simulink model "HarnessModel_BatteryHV"  (R2026a)
settings: Solver=daessc  StopTime=3600
PreLoadFcn:
  | setupHarness_BatteryHV
undefined symbols (not defined in the file or in its folder): Minus, Plus
libraries: nesl_utility x6, fl_lib x5
settings Model: Creator=isaacito  LastModifiedBy=isaacito
settings SimscapeCC: SimscapeNominalValues="[{\"value\":\"1\",\"unit\":\"A\"},{\"value\":\"1\",\"unit\":\"bar\"},{\"value\":\"1\",\"unit\":\"cm^2\"},{\"value\":\"1\",\"unit\":\"cm^3/s\"},{\"value\":\"1\",\"unit\":\"kJ/kg\"},{\"value\":\"1\",\"unit\":\"kW\"},{\"value\":\"1\",\"unit\":\"l\"},{\"value\":\"1\",\"unit\":\"N\"},{\"value\":\"1\",\"unit\":\"N*m\"},{\"value\":\"1\",\"unit\":\"V\"}]"  SimscapeLogSimulationStatistics=on  SimscapeLogLimitData=off  SimscapeLogDataHistory=5000.0

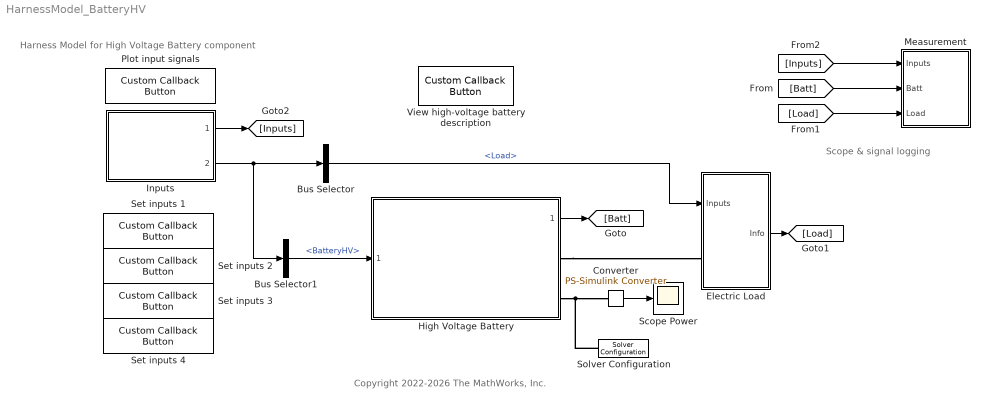
== system HarnessModel_BatteryHV ==
  note: Harness Model for High Voltage Battery component
  note: Copyright 2022-2026 The MathWorks, Inc.
  note: Scope & signal logging
  Bus Selector : BusSelector  OutputSignals=Load
  Bus Selector1 : BusSelector  OutputSignals=BatteryHV
  Converter : nesl_utility/PS-Simulink Converter  PhysicalDomain=network_engine_domain  SubClassName=ps_output  LeftPortType=input  RightPortType=output  PseudoPeriodic=off  Frequencies=[]  VectorFormat=inherit  Unit=kW  AffineConversion=off
  Electric Load : Subsystem
  High Voltage Battery : Subsystem  ReferencedSubsystem=BatteryHV_Basic_refsub
      settings: OpenFcn=|
      | % Look under mask:
      | open_system(gcb, "force")
  Inputs : Subsystem  ReferencedSubsystem=Inputs_BatteryHV_refsub
      settings: OpenFcn="open_system(gcb, \"force\")"
  Measurement : Subsystem
  Plot input signals : CustomCallbackButton  Configuration="{\"components\":[{\"name\":\"BackgroundImageComponent\",\"settings\":{\"image\":{\"size\":[0,0],\"src\":\"default\",\"srcOrientation\":\"Right\"},\"position\":[0,0,1,1]}},{\"name\":\"ButtonStateComponent\",\"settings\":{\"buttonType\":\"momentary\",\"clickFcn\":\"bevutil1.SignalUtil.plotLookupTable1DBlocks(bdroot+\\\"\\/Inputs\\\", Blocks=[\\\"\\/Load current\\\"; \\\"\\/Heat flow\\\"], DivisionType=\\\"InterpolationInterval\\\", InterpolationInterval=0.2)\",\"onValue\":1,\"position\":[0,0,1,1],\"pressDelay\":\"500\",\"pressFcn\":\"\",\"repeatInterval\":\"0\",\"states\":[{\"horizontalAlignment\":\"center\",\"image\":{\"position\":[0,0,1,1],\"size\":[1,1],\"src\":\"default\",\"srcOrientation\":\"Right\"},\"label\":{\"color\":[0.01176470588,0.01176470588,0.01176470588,1],\"icon\":{\"size\":[0,0],\"src\":\"default\",\"srcOrientation\":\"Right\"},\"iconOffset\":0,\"iconPlacement\":\"left\",\"opacity\":1,\"show\":true,\"text\":{\"content\":\"Plot inputs\",\"font\":\"Helvetica\"}},\"labelOffset\":[0,0],\"verticalAlignment\":\"middle\"},{\"horizontalAlignment\":\"center\",\"image\":{\"position\":[0,0,1,1],\"size\":[1,1],\"src\":\"default\",\"srcOrientation\":\"Right\"},\"label\":{\"color\":[0.01176470588,0.01176470588,0.01176470588,1],\"icon\":{\"size\":[0,0],\"src\":\"default\",\"srcOrientation\":\"Right\"},\"iconOffset\":0,\"iconPlacement\":\"left\",\"opacity\":1,\"show\":true,\"text\":{\"content\":\"Plot inputs\",\"font\":\"Helvetica\"}},\"labelOffset\":[0,0],\"verticalAlignment\":\"middle\"},{\"horizontalAlignment\":\"center\",\"image\":{\"position\":[0,0,1,1],\"size\":[1,1],\"src\":\"default\",\"srcOrientation\":\"Right\"},\"label\":{\"color\":[0.01176470588,0.01176470588,0.01176470588,1],\"icon\":{\"size\":[0,0],\"src\":\"default\",\"srcOrientation\":\"Right\"},\"iconOffset\":0,\"iconPlacement\":\"left\",\"opacity\":1,\"show\":true,\"text\":{\"content\":\"Plot inputs\",\"font\":\"Helvetica\"}},\"labelOffset\":[0,0],\"verticalAlignment\":\"middle\"},{\"horizontalAlignment\":\"center\",\"image\":{\"position\":[0,0,1,1],\"size\":[1,1],\"src\":\"default\",\"srcOrientation\":\"Right\"},\"label\":{\"color\":[0.01176470588,0.01176470588,0.01176470588,1],\"icon\":{\"size\":[0,0],\"src\":\"default\",\"srcOrientation\":\"Right\"},\"iconOffset\":0,\"iconPlacement\":\"left\",\"opacity\":1,\"show\":true,\"text\":{\"content\":\"Plot inputs\",\"font\":\"Helvetica\"}},\"labelOffset\":[0,0],\"verticalAlignment\":\"middle\"}]}},{\"name\":\"ForegroundImageComponent\",\"settings\":{\"image\":{\"size\":[0,0],\"src\":\"default\",\"srcOrientation\":\"Right\"},\"isForeground\":1,\"position\":[0,0,1,1]}}],\"derived\":{\"blockParameters\":{\"AutoActivate\":true,\"ButtonText\":\"Plot inputs\",\"ButtonType\":\"Momentary\",\"ClickFcn\":\"bevutil1.SignalUtil.plotLookupTable1DBlocks(bdroot+\\\"\\/Inputs\\\", Blocks=[\\\"\\/Load current\\\"; \\\"\\/Heat flow\\\"], DivisionType=\\\"InterpolationInterval\\\", InterpolationInterval=0.2)\",\"OnValue\":1,\"PressDelay\":\"500\",\"PressFcn\":\"\",\"RepeatInterval\":\"0\",\"fixedAspectRatio\":\"off\"}},\"settings\":{\"BindingType\":\"standalone\",\"autoActivate\":true,\"backgroundColor\":[244,244,244,1],\"backgroundOffset\":0.2,\"backgroundOpacity\":1,\"fixedAspectRatio\":\"off\",\"foregroundColor\":[0.01176470588,0.01176470588,0.01176470588,1],\"migratedFromLegacy\":true,\"useBackgroundColor\":true,\"variant\":\"callback\",\"version\":\"R2025a\"},\"type\":\"Button\"}"  CustomBackgroundColor="{\"color\":[0.9568627451,0.9568627451,0.9568627451],\"show\":true}"
  Scope Power : Scope
      settings: ActiveDisplayYMinimum=-3.3202715007040107  ActiveDisplayYMaximum=7.2203137029230895
  Set inputs 1 : CustomCallbackButton  Configuration="{\"components\":[{\"name\":\"BackgroundImageComponent\",\"settings\":{\"image\":{\"size\":[0,0],\"src\":\"default\",\"srcOrientation\":\"Right\"},\"position\":[0,0,1,1]}},{\"name\":\"ButtonStateComponent\",\"settings\":{\"buttonType\":\"momentary\",\"clickFcn\":\"BatteryHV_Basic_params\\nset_param(gcs, StopTime=\\\"3600\\\")\\n\\ndisp(\\\"Loading inputs: <a href=\\\"\\\"matlab:edit('LoadInputs_BatteryHV_Constant')\\\"\\\">Constant<\\/a>\\\")\\nLoadInputs_BatteryHV_Constant\\n\",\"onValue\":1,\"position\":[0,0,1,1],\"pressDelay\":\"500\",\"pressFcn\":\"\",\"repeatInterval\":\"0\",\"states\":[{\"horizontalAlignment\":\"center\",\"image\":{\"position\":[0,0,1,1],\"size\":[1,1],\"src\":\"default\",\"srcOrientation\":\"Right\"},\"label\":{\"color\":[0.01176470588,0.01176470588,0.01176470588,1],\"icon\":{\"size\":[0,0],\"src\":\"default\",\"srcOrientation\":\"Right\"},\"iconOffset\":0,\"iconPlacement\":\"left\",\"opacity\":1,\"show\":true,\"text\":{\"content\":\"Constant\",\"font\":\"Helvetica\"}},\"labelOffset\":[0,0],\"verticalAlignment\":\"middle\"},{\"horizontalAlignment\":\"center\",\"image\":{\"position\":[0,0,1,1],\"size\":[1,1],\"src\":\"default\",\"srcOrientation\":\"Right\"},\"label\":{\"color\":[0.01176470588,0.01176470588,0.01176470588,1],\"icon\":{\"size\":[0,0],\"src\":\"default\",\"srcOrientation\":\"Right\"},\"iconOffset\":0,\"iconPlacement\":\"left\",\"opacity\":1,\"show\":true,\"text\":{\"content\":\"Constant\",\"font\":\"Helvetica\"}},\"labelOffset\":[0,0],\"verticalAlignment\":\"middle\"},{\"horizontalAlignment\":\"center\",\"image\":{\"position\":[0,0,1,1],\"size\":[1,1],\"src\":\"default\",\"srcOrientation\":\"Right\"},\"label\":{\"color\":[0.01176470588,0.01176470588,0.01176470588,1],\"icon\":{\"size\":[0,0],\"src\":\"default\",\"srcOrientation\":\"Right\"},\"iconOffset\":0,\"iconPlacement\":\"left\",\"opacity\":1,\"show\":true,\"text\":{\"content\":\"Constant\",\"font\":\"Helvetica\"}},\"labelOffset\":[0,0],\"verticalAlignment\":\"middle\"},{\"horizontalAlignment\":\"center\",\"image\":{\"position\":[0,0,1,1],\"size\":[1,1],\"src\":\"default\",\"srcOrientation\":\"Right\"},\"label\":{\"color\":[0.01176470588,0.01176470588,0.01176470588,1],\"icon\":{\"size\":[0,0],\"src\":\"default\",\"srcOrientation\":\"Right\"},\"iconOffset\":0,\"iconPlacement\":\"left\",\"opacity\":1,\"show\":true,\"text\":{\"content\":\"Constant\",\"font\":\"Helvetica\"}},\"labelOffset\":[0,0],\"verticalAlignment\":\"middle\"}]}},{\"name\":\"ForegroundImageComponent\",\"settings\":{\"image\":{\"size\":[0,0],\"src\":\"default\",\"srcOrientation\":\"Right\"},\"isForeground\":1,\"position\":[0,0,1,1]}}],\"derived\":{\"blockParameters\":{\"AutoActivate\":true,\"ButtonText\":\"Constant\",\"ButtonType\":\"Momentary\",\"ClickFcn\":\"BatteryHV_Basic_params\\nset_param(gcs, StopTime=\\\"3600\\\")\\n\\ndisp(\\\"Loading inputs: <a href=\\\"\\\"matlab:edit('LoadInputs_BatteryHV_Constant')\\\"\\\">Constant<\\/a>\\\")\\nLoadInputs_BatteryHV_Constant\\n\",\"OnValue\":1,\"PressDelay\":\"500\",\"PressFcn\":\"\",\"RepeatInterval\":\"0\",\"fixedAspectRatio\":\"off\"}},\"settings\":{\"BindingType\":\"standalone\",\"autoActivate\":true,\"backgroundColor\":[244,244,244,1],\"backgroundOffset\":0.2,\"backgroundOpacity\":1,\"fixedAspectRatio\":\"off\",\"foregroundColor\":[0.01176470588,0.01176470588,0.01176470588,1],\"migratedFromLegacy\":true,\"useBackgroundColor\":true,\"variant\":\"callback\",\"version\":\"R2025a\"},\"type\":\"Button\"}"  CustomBackgroundColor="{\"color\":[0.9568627451,0.9568627451,0.9568627451],\"show\":true}"
  Set inputs 2 : CustomCallbackButton  Configuration="{\"components\":[{\"name\":\"BackgroundImageComponent\",\"settings\":{\"image\":{\"size\":[0,0],\"src\":\"default\",\"srcOrientation\":\"Right\"},\"position\":[0,0,1,1]}},{\"name\":\"ButtonStateComponent\",\"settings\":{\"buttonType\":\"momentary\",\"clickFcn\":\"BatteryHV_Basic_params\\nset_param(gcs, StopTime=\\\"3600\\\")\\n\\ndisp(\\\"Loading inputs: <a href=\\\"\\\"matlab:edit('LoadInputs_BatteryHV_Charge')\\\"\\\">Charge<\\/a>\\\")\\nLoadInputs_BatteryHV_Charge\\n\",\"onValue\":1,\"position\":[0,0,1,1],\"pressDelay\":\"500\",\"pressFcn\":\"\",\"repeatInterval\":\"0\",\"states\":[{\"horizontalAlignment\":\"center\",\"image\":{\"position\":[0,0,1,1],\"size\":[1,1],\"src\":\"default\",\"srcOrientation\":\"Right\"},\"label\":{\"color\":[0.01176470588,0.01176470588,0.01176470588,1],\"icon\":{\"size\":[0,0],\"src\":\"default\",\"srcOrientation\":\"Right\"},\"iconOffset\":0,\"iconPlacement\":\"left\",\"opacity\":1,\"show\":true,\"text\":{\"content\":\"Charge\",\"font\":\"Helvetica\"}},\"labelOffset\":[0,0],\"verticalAlignment\":\"middle\"},{\"horizontalAlignment\":\"center\",\"image\":{\"position\":[0,0,1,1],\"size\":[1,1],\"src\":\"default\",\"srcOrientation\":\"Right\"},\"label\":{\"color\":[0.01176470588,0.01176470588,0.01176470588,1],\"icon\":{\"size\":[0,0],\"src\":\"default\",\"srcOrientation\":\"Right\"},\"iconOffset\":0,\"iconPlacement\":\"left\",\"opacity\":1,\"show\":true,\"text\":{\"content\":\"Charge\",\"font\":\"Helvetica\"}},\"labelOffset\":[0,0],\"verticalAlignment\":\"middle\"},{\"horizontalAlignment\":\"center\",\"image\":{\"position\":[0,0,1,1],\"size\":[1,1],\"src\":\"default\",\"srcOrientation\":\"Right\"},\"label\":{\"color\":[0.01176470588,0.01176470588,0.01176470588,1],\"icon\":{\"size\":[0,0],\"src\":\"default\",\"srcOrientation\":\"Right\"},\"iconOffset\":0,\"iconPlacement\":\"left\",\"opacity\":1,\"show\":true,\"text\":{\"content\":\"Charge\",\"font\":\"Helvetica\"}},\"labelOffset\":[0,0],\"verticalAlignment\":\"middle\"},{\"horizontalAlignment\":\"center\",\"image\":{\"position\":[0,0,1,1],\"size\":[1,1],\"src\":\"default\",\"srcOrientation\":\"Right\"},\"label\":{\"color\":[0.01176470588,0.01176470588,0.01176470588,1],\"icon\":{\"size\":[0,0],\"src\":\"default\",\"srcOrientation\":\"Right\"},\"iconOffset\":0,\"iconPlacement\":\"left\",\"opacity\":1,\"show\":true,\"text\":{\"content\":\"Charge\",\"font\":\"Helvetica\"}},\"labelOffset\":[0,0],\"verticalAlignment\":\"middle\"}]}},{\"name\":\"ForegroundImageComponent\",\"settings\":{\"image\":{\"size\":[0,0],\"src\":\"default\",\"srcOrientation\":\"Right\"},\"isForeground\":1,\"position\":[0,0,1,1]}}],\"derived\":{\"blockParameters\":{\"AutoActivate\":true,\"ButtonText\":\"Charge\",\"ButtonType\":\"Momentary\",\"ClickFcn\":\"BatteryHV_Basic_params\\nset_param(gcs, StopTime=\\\"3600\\\")\\n\\ndisp(\\\"Loading inputs: <a href=\\\"\\\"matlab:edit('LoadInputs_BatteryHV_Charge')\\\"\\\">Charge<\\/a>\\\")\\nLoadInputs_BatteryHV_Charge\\n\",\"OnValue\":1,\"PressDelay\":\"500\",\"PressFcn\":\"\",\"RepeatInterval\":\"0\",\"fixedAspectRatio\":\"off\"}},\"settings\":{\"BindingType\":\"standalone\",\"autoActivate\":true,\"backgroundColor\":[244,244,244,1],\"backgroundOffset\":0.2,\"backgroundOpacity\":1,\"fixedAspectRatio\":\"off\",\"foregroundColor\":[0.01176470588,0.01176470588,0.01176470588,1],\"migratedFromLegacy\":true,\"useBackgroundColor\":true,\"variant\":\"callback\",\"version\":\"R2025a\"},\"type\":\"Button\"}"  CustomBackgroundColor="{\"color\":[0.9568627451,0.9568627451,0.9568627451],\"show\":true}"
  Set inputs 3 : CustomCallbackButton  Configuration="{\"components\":[{\"name\":\"BackgroundImageComponent\",\"settings\":{\"image\":{\"size\":[0,0],\"src\":\"default\",\"srcOrientation\":\"Right\"},\"position\":[0,0,1,1]}},{\"name\":\"ButtonStateComponent\",\"settings\":{\"buttonType\":\"momentary\",\"clickFcn\":\"BatteryHV_Basic_params\\nset_param(gcs, StopTime=\\\"3600\\\")\\n\\ndisp(\\\"Loading inputs: <a href=\\\"\\\"matlab:edit('LoadInputs_BatteryHV_Discharge')\\\"\\\">Discharge<\\/a>\\\")\\nLoadInputs_BatteryHV_Discharge\\n\",\"onValue\":1,\"position\":[0,0,1,1],\"pressDelay\":\"500\",\"pressFcn\":\"\",\"repeatInterval\":\"0\",\"states\":[{\"horizontalAlignment\":\"center\",\"image\":{\"position\":[0,0,1,1],\"size\":[1,1],\"src\":\"default\",\"srcOrientation\":\"Right\"},\"label\":{\"color\":[0.01176470588,0.01176470588,0.01176470588,1],\"icon\":{\"size\":[0,0],\"src\":\"default\",\"srcOrientation\":\"Right\"},\"iconOffset\":0,\"iconPlacement\":\"left\",\"opacity\":1,\"show\":true,\"text\":{\"content\":\"Discharge\",\"font\":\"Helvetica\"}},\"labelOffset\":[0,0],\"verticalAlignment\":\"middle\"},{\"horizontalAlignment\":\"center\",\"image\":{\"position\":[0,0,1,1],\"size\":[1,1],\"src\":\"default\",\"srcOrientation\":\"Right\"},\"label\":{\"color\":[0.01176470588,0.01176470588,0.01176470588,1],\"icon\":{\"size\":[0,0],\"src\":\"default\",\"srcOrientation\":\"Right\"},\"iconOffset\":0,\"iconPlacement\":\"left\",\"opacity\":1,\"show\":true,\"text\":{\"content\":\"Discharge\",\"font\":\"Helvetica\"}},\"labelOffset\":[0,0],\"verticalAlignment\":\"middle\"},{\"horizontalAlignment\":\"center\",\"image\":{\"position\":[0,0,1,1],\"size\":[1,1],\"src\":\"default\",\"srcOrientation\":\"Right\"},\"label\":{\"color\":[0.01176470588,0.01176470588,0.01176470588,1],\"icon\":{\"size\":[0,0],\"src\":\"default\",\"srcOrientation\":\"Right\"},\"iconOffset\":0,\"iconPlacement\":\"left\",\"opacity\":1,\"show\":true,\"text\":{\"content\":\"Discharge\",\"font\":\"Helvetica\"}},\"labelOffset\":[0,0],\"verticalAlignment\":\"middle\"},{\"horizontalAlignment\":\"center\",\"image\":{\"position\":[0,0,1,1],\"size\":[1,1],\"src\":\"default\",\"srcOrientation\":\"Right\"},\"label\":{\"color\":[0.01176470588,0.01176470588,0.01176470588,1],\"icon\":{\"size\":[0,0],\"src\":\"default\",\"srcOrientation\":\"Right\"},\"iconOffset\":0,\"iconPlacement\":\"left\",\"opacity\":1,\"show\":true,\"text\":{\"content\":\"Discharge\",\"font\":\"Helvetica\"}},\"labelOffset\":[0,0],\"verticalAlignment\":\"middle\"}]}},{\"name\":\"ForegroundImageComponent\",\"settings\":{\"image\":{\"size\":[0,0],\"src\":\"default\",\"srcOrientation\":\"Right\"},\"isForeground\":1,\"position\":[0,0,1,1]}}],\"derived\":{\"blockParameters\":{\"AutoActivate\":true,\"ButtonText\":\"Discharge\",\"ButtonType\":\"Momentary\",\"ClickFcn\":\"BatteryHV_Basic_params\\nset_param(gcs, StopTime=\\\"3600\\\")\\n\\ndisp(\\\"Loading inputs: <a href=\\\"\\\"matlab:edit('LoadInputs_BatteryHV_Discharge')\\\"\\\">Discharge<\\/a>\\\")\\nLoadInputs_BatteryHV_Discharge\\n\",\"OnValue\":1,\"PressDelay\":\"500\",\"PressFcn\":\"\",\"RepeatInterval\":\"0\",\"fixedAspectRatio\":\"off\"}},\"settings\":{\"BindingType\":\"standalone\",\"autoActivate\":true,\"backgroundColor\":[244,244,244,1],\"backgroundOffset\":0.2,\"backgroundOpacity\":1,\"fixedAspectRatio\":\"off\",\"foregroundColor\":[0.01176470588,0.01176470588,0.01176470588,1],\"migratedFromLegacy\":true,\"useBackgroundColor\":true,\"variant\":\"callback\",\"version\":\"R2025a\"},\"type\":\"Button\"}"  CustomBackgroundColor="{\"color\":[0.9568627451,0.9568627451,0.9568627451],\"show\":true}"
  Set inputs 4 : CustomCallbackButton  Configuration="{\"components\":[{\"name\":\"BackgroundImageComponent\",\"settings\":{\"image\":{\"size\":[0,0],\"src\":\"default\",\"srcOrientation\":\"Right\"},\"position\":[0,0,1,1]}},{\"name\":\"ButtonStateComponent\",\"settings\":{\"buttonType\":\"momentary\",\"clickFcn\":\"BatteryHV_Basic_params\\n\\ndisp(\\\"Loading inputs: <a href=\\\"\\\"matlab:edit('LoadInputs_BatteryHV_Random')\\\"\\\">Random<\\/a>\\\")\\nLoadInputs_BatteryHV_Random\\n\\ntmp_stop_time = get_param(bdroot+\\\"\\/Inputs\\/Load current\\\", \\\"value@BreakpointsForDimension1\\\");\\nset_param(bdroot, StopTime=num2str(tmp_stop_time(end)) )\\ndisp(\\\"Stop time: \\\" + tmp_stop_time(end))\\nclear tmp_stop_time\\n\",\"onValue\":1,\"position\":[0,0,1,1],\"pressDelay\":\"500\",\"pressFcn\":\"\",\"repeatInterval\":\"0\",\"states\":[{\"horizontalAlignment\":\"center\",\"image\":{\"position\":[0,0,1,1],\"size\":[1,1],\"src\":\"default\",\"srcOrientation\":\"Right\"},\"label\":{\"color\":[0.01176470588,0.01176470588,0.01176470588,1],\"icon\":{\"size\":[0,0],\"src\":\"default\",\"srcOrientation\":\"Right\"},\"iconOffset\":0,\"iconPlacement\":\"left\",\"opacity\":1,\"show\":true,\"text\":{\"content\":\"Random\",\"font\":\"Helvetica\"}},\"labelOffset\":[0,0],\"verticalAlignment\":\"middle\"},{\"horizontalAlignment\":\"center\",\"image\":{\"position\":[0,0,1,1],\"size\":[1,1],\"src\":\"default\",\"srcOrientation\":\"Right\"},\"label\":{\"color\":[0.01176470588,0.01176470588,0.01176470588,1],\"icon\":{\"size\":[0,0],\"src\":\"default\",\"srcOrientation\":\"Right\"},\"iconOffset\":0,\"iconPlacement\":\"left\",\"opacity\":1,\"show\":true,\"text\":{\"content\":\"Random\",\"font\":\"Helvetica\"}},\"labelOffset\":[0,0],\"verticalAlignment\":\"middle\"},{\"horizontalAlignment\":\"center\",\"image\":{\"position\":[0,0,1,1],\"size\":[1,1],\"src\":\"default\",\"srcOrientation\":\"Right\"},\"label\":{\"color\":[0.01176470588,0.01176470588,0.01176470588,1],\"icon\":{\"size\":[0,0],\"src\":\"default\",\"srcOrientation\":\"Right\"},\"iconOffset\":0,\"iconPlacement\":\"left\",\"opacity\":1,\"show\":true,\"text\":{\"content\":\"Random\",\"font\":\"Helvetica\"}},\"labelOffset\":[0,0],\"verticalAlignment\":\"middle\"},{\"horizontalAlignment\":\"center\",\"image\":{\"position\":[0,0,1,1],\"size\":[1,1],\"src\":\"default\",\"srcOrientation\":\"Right\"},\"label\":{\"color\":[0.01176470588,0.01176470588,0.01176470588,1],\"icon\":{\"size\":[0,0],\"src\":\"default\",\"srcOrientation\":\"Right\"},\"iconOffset\":0,\"iconPlacement\":\"left\",\"opacity\":1,\"show\":true,\"text\":{\"content\":\"Random\",\"font\":\"Helvetica\"}},\"labelOffset\":[0,0],\"verticalAlignment\":\"middle\"}]}},{\"name\":\"ForegroundImageComponent\",\"settings\":{\"image\":{\"size\":[0,0],\"src\":\"default\",\"srcOrientation\":\"Right\"},\"isForeground\":1,\"position\":[0,0,1,1]}}],\"derived\":{\"blockParameters\":{\"AutoActivate\":true,\"ButtonText\":\"Random\",\"ButtonType\":\"Momentary\",\"ClickFcn\":\"BatteryHV_Basic_params\\n\\ndisp(\\\"Loading inputs: <a href=\\\"\\\"matlab:edit('LoadInputs_BatteryHV_Random')\\\"\\\">Random<\\/a>\\\")\\nLoadInputs_BatteryHV_Random\\n\\ntmp_stop_time = get_param(bdroot+\\\"\\/Inputs\\/Load current\\\", \\\"value@BreakpointsForDimension1\\\");\\nset_param(bdroot, StopTime=num2str(tmp_stop_time(end)) )\\ndisp(\\\"Stop time: \\\" + tmp_stop_time(end))\\nclear tmp_stop_time\\n\",\"OnValue\":1,\"PressDelay\":\"500\",\"PressFcn\":\"\",\"RepeatInterval\":\"0\",\"fixedAspectRatio\":\"off\"}},\"settings\":{\"BindingType\":\"standalone\",\"autoActivate\":true,\"backgroundColor\":[244,244,244,1],\"backgroundOffset\":0.2,\"backgroundOpacity\":1,\"fixedAspectRatio\":\"off\",\"foregroundColor\":[0.01176470588,0.01176470588,0.01176470588,1],\"migratedFromLegacy\":true,\"useBackgroundColor\":true,\"variant\":\"callback\",\"version\":\"R2025a\"},\"type\":\"Button\"}"  CustomBackgroundColor="{\"color\":[0.9568627451,0.9568627451,0.9568627451],\"show\":true}"
  Solver Configuration : nesl_utility/Solver Configuration  PhysicalDomain=network_engine_domain  SubClassName=solver  LeftPortType=input  RightPortType=generic  Tones=[]  Harmonics=[]  SimulateNoise=off  Profile=off  UseLocalSampling=off  EnableSwitchedLinearOptims=on  FrequencyDomain=off  UseCCode=off  RelTol=0.001  AbsTol=0.001  MinStep=1e-09  ToWorkspace=off  RevertToSquareIcSolve=off  NumHomotopyIterations=100  PhasorMode=off  PhasorModeNumHarmonics=1  ConsistencySolver=NEWTON_FTOL  CanonicalOrdering=UNORDERED  OptimizeIntermediates=UNOPTIMIZED  IndexReductionMethod=DerivativeReplacement  DoDC=off  ResidualTolerance=1e-09  ConsistencyTolSource=GLOBAL  ConsistencyAbsTol=0.001  ConsistencyRelTol=0.001  ConsistencyTolFactor=0.001  UseLocalSolver=off  LocalSolverChoice=NE_BACKWARD_EULER_ADVANCER  ResolveIndetEquations=on  FunctionEvalNumThread=1  LocalSolverSampleTime=0.001  DoFixedCost=off  MaxNonlinIter=3  MaxModeIter=2  ComputeImpulses=off  ImpulseIterations=2  LinearAlgebra=auto  LinearAlgebraNumThread=0  EquationFormulation=NE_TIME_EF  DelaysMemoryBudget=1024  AutomaticFiltering=on  FilteringTimeConstant=0.001  PartitionStorageMethod=AS_NEEDED  PartitionMemoryBudget=1024  PartitionMethod=ROBUST  MultibodyUseLocalSolver=off  MultibodyLocalSolverChoice=ODE1  MultibodyLocalSolverSampleTime=0.001
      settings: AttributesFormatString=Local solver: %<UseLocalSolver>
  View high-voltage battery description : CustomCallbackButton  Configuration="{\"components\":[{\"name\":\"BackgroundImageComponent\",\"settings\":{\"image\":{\"size\":[0,0],\"src\":\"default\",\"srcOrientation\":\"Right\"},\"position\":[0,0,1,1]}},{\"name\":\"ButtonStateComponent\",\"settings\":{\"buttonType\":\"momentary\",\"clickFcn\":\"web(\\\"BatteryHV_Description.html\\\")\",\"onValue\":1,\"position\":[0,0,1,1],\"pressDelay\":\"500\",\"pressFcn\":\"\",\"repeatInterval\":\"0\",\"states\":[{\"horizontalAlignment\":\"center\",\"image\":{\"position\":[0,0,1,1],\"size\":[1,1],\"src\":\"default\",\"srcOrientation\":\"Right\"},\"label\":{\"color\":[0.01176470588,0.01176470588,0.01176470588,1],\"icon\":{\"size\":[0,0],\"src\":\"default\",\"srcOrientation\":\"Right\"},\"iconOffset\":0,\"iconPlacement\":\"left\",\"opacity\":1,\"show\":true,\"text\":{\"content\":\"Open page\",\"font\":\"Helvetica\"}},\"labelOffset\":[0,0],\"verticalAlignment\":\"middle\"},{\"horizontalAlignment\":\"center\",\"image\":{\"position\":[0,0,1,1],\"size\":[1,1],\"src\":\"default\",\"srcOrientation\":\"Right\"},\"label\":{\"color\":[0.01176470588,0.01176470588,0.01176470588,1],\"icon\":{\"size\":[0,0],\"src\":\"default\",\"srcOrientation\":\"Right\"},\"iconOffset\":0,\"iconPlacement\":\"left\",\"opacity\":1,\"show\":true,\"text\":{\"content\":\"Open page\",\"font\":\"Helvetica\"}},\"labelOffset\":[0,0],\"verticalAlignment\":\"middle\"},{\"horizontalAlignment\":\"center\",\"image\":{\"position\":[0,0,1,1],\"size\":[1,1],\"src\":\"default\",\"srcOrientation\":\"Right\"},\"label\":{\"color\":[0.01176470588,0.01176470588,0.01176470588,1],\"icon\":{\"size\":[0,0],\"src\":\"default\",\"srcOrientation\":\"Right\"},\"iconOffset\":0,\"iconPlacement\":\"left\",\"opacity\":1,\"show\":true,\"text\":{\"content\":\"Open page\",\"font\":\"Helvetica\"}},\"labelOffset\":[0,0],\"verticalAlignment\":\"middle\"},{\"horizontalAlignment\":\"center\",\"image\":{\"position\":[0,0,1,1],\"size\":[1,1],\"src\":\"default\",\"srcOrientation\":\"Right\"},\"label\":{\"color\":[0.01176470588,0.01176470588,0.01176470588,1],\"icon\":{\"size\":[0,0],\"src\":\"default\",\"srcOrientation\":\"Right\"},\"iconOffset\":0,\"iconPlacement\":\"left\",\"opacity\":1,\"show\":true,\"text\":{\"content\":\"Open page\",\"font\":\"Helvetica\"}},\"labelOffset\":[0,0],\"verticalAlignment\":\"middle\"}]}},{\"name\":\"ForegroundImageComponent\",\"settings\":{\"image\":{\"size\":[0,0],\"src\":\"default\",\"srcOrientation\":\"Right\"},\"isForeground\":1,\"position\":[0,0,1,1]}}],\"derived\":{\"blockParameters\":{\"AutoActivate\":true,\"ButtonText\":\"Open page\",\"ButtonType\":\"Momentary\",\"ClickFcn\":\"web(\\\"BatteryHV_Description.html\\\")\",\"OnValue\":1,\"PressDelay\":\"500\",\"PressFcn\":\"\",\"RepeatInterval\":\"0\",\"fixedAspectRatio\":\"off\"}},\"settings\":{\"BindingType\":\"standalone\",\"autoActivate\":true,\"backgroundColor\":[244,244,244,1],\"backgroundOffset\":0.2,\"backgroundOpacity\":1,\"fixedAspectRatio\":\"off\",\"foregroundColor\":[0.01176470588,0.01176470588,0.01176470588,1],\"migratedFromLegacy\":true,\"useBackgroundColor\":true,\"variant\":\"callback\",\"version\":\"R2025a\"},\"type\":\"Button\"}"  CustomBackgroundColor="{\"color\":[0.9568627450980393,0.9568627450980393,0.9568627450980393],\"show\":true}"
  wires:
  High Voltage Battery/1 -> [Batt]
  [Batt] -> Measurement/2(Batt)
  Electric Load/1(Info) -> [Load]
  [Load] -> Measurement/3(Load)
  [Inputs] -> Measurement/1(Inputs)
  Inputs/1 -> [Inputs]
  Inputs/2 -> Bus Selector/1, Bus Selector1/1
  Bus Selector/1 -> Electric Load/1(Inputs)  "<Load>"
  Bus Selector1/1 -> High Voltage Battery/1  "<BatteryHV>"
  Converter/1 -> Scope Power/1
  connections:
  High Voltage Battery/RConn1 -- Electric Load/LConn1
  High Voltage Battery/RConn2 -- Solver Configuration/RConn1 -- Converter/LConn1

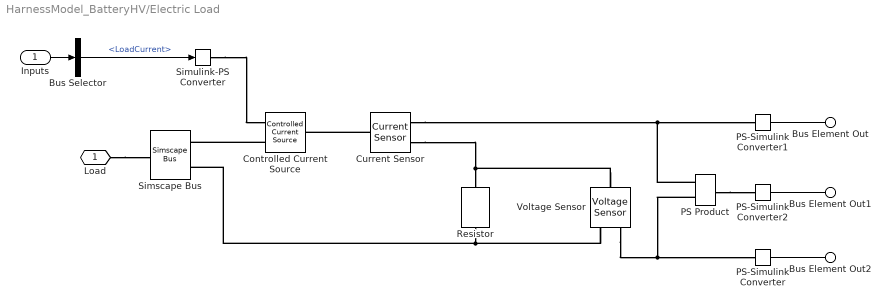
== system HarnessModel_BatteryHV/Electric Load ==
  Inputs : Inport
  Bus Selector : BusSelector  OutputSignals=LoadCurrent
  Controlled Current Source : fl_lib/Electrical/Electrical Sources/Controlled Current Source
  Current Sensor : fl_lib/Electrical/Electrical Sensors/Current Sensor
  PS Product : fl_lib/Physical Signals/Functions/PS Product
  PS-Simulink Converter : nesl_utility/PS-Simulink Converter  PhysicalDomain=network_engine_domain  SubClassName=ps_output  LeftPortType=input  RightPortType=output  PseudoPeriodic=off  Frequencies=[]  VectorFormat=inherit  Unit=V  AffineConversion=off
  PS-Simulink Converter1 : nesl_utility/PS-Simulink Converter  PhysicalDomain=network_engine_domain  SubClassName=ps_output  LeftPortType=input  RightPortType=output  PseudoPeriodic=off  Frequencies=[]  VectorFormat=inherit  Unit=A  AffineConversion=off
  PS-Simulink Converter2 : nesl_utility/PS-Simulink Converter  PhysicalDomain=network_engine_domain  SubClassName=ps_output  LeftPortType=input  RightPortType=output  PseudoPeriodic=off  Frequencies=[]  VectorFormat=inherit  Unit=kW  AffineConversion=off
  Resistor : fl_lib/Electrical/Electrical Elements/Resistor  R=1 Ohm  i_specify=off  i_priority=None  i=0 A  i_nominal_specify=off  i_nominal_value=1  i_nominal_unit=A  v_specify=off  v_priority=None  v=0 V  v_nominal_specify=off  v_nominal_value=1  v_nominal_unit=V
  Simscape Bus : SimscapeBus  HierarchyStrings=Plus;Minus  ConnectionType=Bus: Bus_HighVoltage
  Simulink-PS Converter : nesl_utility/Simulink-PS Converter  PhysicalDomain=network_engine_domain  SubClassName=ps_input  LeftPortType=input  RightPortType=output  PseudoPeriodic=off  Frequencies=[]  NoiseDistribution=none  NoiseParameters=[]  Unit=A  AffineConversion=off  FilteringAndDerivatives=provide  SimscapeFilterOrder=1  InputFilterTimeConstant=0.001  UdotUserProvided=0
  Voltage Sensor : fl_lib/Electrical/Electrical Sensors/Voltage Sensor
  Load : PMIOPort  Side=Left
  Bus Element Out : Outport  PortName=Info  Element=Curr
  Bus Element Out1 : Outport  PortName=Info  Element=Pwr
  Bus Element Out2 : Outport  PortName=Info  Element=V
  wires:
  PS-Simulink Converter1/1 -> Bus Element Out/1
  PS-Simulink Converter2/1 -> Bus Element Out1/1
  PS-Simulink Converter/1 -> Bus Element Out2/1
  Inputs/1 -> Bus Selector/1
  Bus Selector/1 -> Simulink-PS Converter/1  "<LoadCurrent>"
  connections:
  Load/RConn1 -- Simscape Bus/RConn1
  Controlled Current Source/RConn2 -- Simscape Bus/LConn1
  Resistor/RConn1 -- Voltage Sensor/RConn2 -- Simscape Bus/LConn2
  Simulink-PS Converter/RConn1 -- Controlled Current Source/RConn1
  Current Sensor/LConn1 -- Controlled Current Source/LConn1
  Current Sensor/RConn2 -- Voltage Sensor/LConn1 -- Resistor/LConn1
  Voltage Sensor/RConn1 -- PS Product/LConn2 -- PS-Simulink Converter/LConn1
  Current Sensor/RConn1 -- PS Product/LConn1 -- PS-Simulink Converter1/LConn1
  PS Product/RConn1 -- PS-Simulink Converter2/LConn1

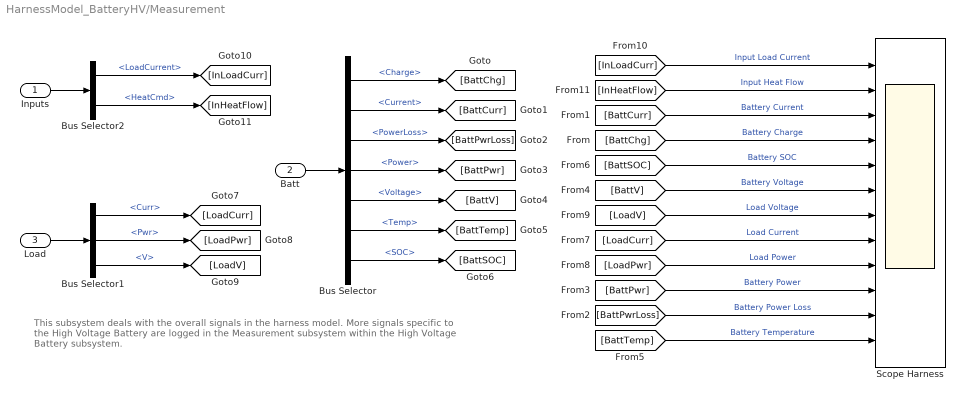
== system HarnessModel_BatteryHV/Measurement ==
  note: This subsystem deals with the overall signals in the harness model.
      | More signals specific to the High Voltage Battery are logged in
      | the Measurement subsystem within the High Voltage Battery subsystem.
  Inputs : Inport
  Batt : Inport  Port=2
  Load : Inport  Port=3
  Bus Selector : BusSelector  OutputSignals=Charge,Current,PowerLoss,Power,Voltage,Temp,SOC
  Bus Selector1 : BusSelector  OutputSignals=Curr,Pwr,V
  Bus Selector2 : BusSelector  OutputSignals=LoadCurrent,HeatCmd
  Scope Harness : Scope  NumInputPorts=12
      settings: ActiveDisplayYMinimum=-10.25  ActiveDisplayYMaximum=22.250000000000004
  wires:
  Batt/1 -> Bus Selector/1
  Bus Selector/1 -> [BattChg]  "<Charge>"
  Bus Selector/2 -> [BattCurr]  "<Current>"
  Bus Selector/3 -> [BattPwrLoss]  "<PowerLoss>"
  Bus Selector/4 -> [BattPwr]  "<Power>"
  Bus Selector/5 -> [BattV]  "<Voltage>"
  Bus Selector/6 -> [BattTemp]  "<Temp>"
  Bus Selector/7 -> [BattSOC]  "<SOC>"
  Load/1 -> Bus Selector1/1
  Bus Selector1/1 -> [LoadCurr]  "<Curr>"
  Bus Selector1/2 -> [LoadPwr]  "<Pwr>"
  Bus Selector1/3 -> [LoadV]  "<V>"
  [BattCurr] -> Scope Harness/3  "Battery Current"
  [BattChg] -> Scope Harness/4  "Battery Charge"
  [BattSOC] -> Scope Harness/5  "Battery SOC"
  [BattV] -> Scope Harness/6  "Battery Voltage"
  [LoadV] -> Scope Harness/7  "Load Voltage"
  [LoadCurr] -> Scope Harness/8  "Load Current"
  [LoadPwr] -> Scope Harness/9  "Load Power"
  [BattPwr] -> Scope Harness/10  "Battery Power"
  [BattPwrLoss] -> Scope Harness/11  "Battery Power Loss"
  [BattTemp] -> Scope Harness/12  "Battery Temperature"
  Inputs/1 -> Bus Selector2/1
  Bus Selector2/1 -> [InLoadCurr]  "<LoadCurrent>"
  [InLoadCurr] -> Scope Harness/1  "Input Load Current"
  Bus Selector2/2 -> [InHeatFlow]  "<HeatCmd>"
  [InHeatFlow] -> Scope Harness/2  "Input Heat Flow"
